simulink model "qs3_dqn_swingup_v4_ctrl"  (R2025b)
settings: Solver=ode1  StartTime=0.0  StopTime=inf  FixedStep=0.002  RelTol=1e-3  AbsTol=1e-6  EnableMultiTasking=on
undefined symbols (not defined in the file): HIL, qc_get_step_size
libraries: quarc_library x3, simulink_extras x3
settings Model: SimulationMode=external  ExtModeTrigDuration=5000  Creator=MLevis  LastModifiedBy=CPB0
settings SolverCC: AutoScaleAbsTol=off  AlgebraicLoopSolver=TrustRegion  PositivePriorityOrder=on
settings DataIOCC: SaveFormat=Array  SignalLoggingSaveFormat=ModelDataLogs  ReturnWorkspaceOutputs=off
settings OptimizationCC: BlockReduction=off  BooleanDataType=off  OptimizeBlockIOStorage=off  BufferReuse=off  GlobalBufferReuse=off  ExpressionFolding=off  ExpressionDepthLimit=2147483647.0  LocalBlockOutputs=off  InitFltsAndDblsToZero=on  OptimizeDataStoreBuffers=off  BusAssignmentInplaceUpdate=off
settings DebuggingCC: SaveWithParameterizedLinksMsg=none  UnderspecifiedInitializationDetection=Classic  MergeDetectMultiDrivingBlocksExec=none  SignalResolutionControl=TryResolveAllWithWarning  MultiTaskDSMMsg=warning  MultiTaskCondExecSysMsg=none  FcnCallInpInsideContextMsg=warning  UnconnectedInputMsg=warning  UnconnectedOutputMsg=warning  UnconnectedLineMsg=warning  StateNameClashWarn=warning  SFUnexpectedBacktrackingDiag=warning  SFNoUnconditionalDefaultTransitionDiag=warning  SFExecutionAtInitializationDiag=none  ArithmeticOperatorsInVariantConditions=warning
settings HardwareCC: TargetHWDeviceType=32-bit Generic
settings ModelReferenceCC: EnableRefExpFcnMdlSchedulingChecks=on  PropagateSignalLabelsOutOfModel=off
settings SFSimCC: SimUseLocalCustomCode=off  CustomCodeUndefinedFunction=UseInterfaceOnly
settings RTWCC: SystemTargetFile=quarc_win64.tlc  TemplateMakefile=quarc_default_tmf  RTWUseLocalCustomCode=off  Toolchain=QUARC win64 | nmake (64-bit Windows)  BuildConfiguration=Faster Runs  GPUComputeCapability=3.5  Description=QUARC Win64 Target Using Toolchain
settings CodeAppCC: StateflowObjectComments=on
settings STFCustomTargetCC: SystemTargetFile=quarc_win64.tlc  UseToolchainInfoCompliant=on
settings GRTTargetCC: ExtMode=on  ExtModeMexFile=quarc_comm  TargetLangStandard=C89/C90 (ANSI)  ParMdlRefBuildCompliant=off  CompOptLevelCompliant=off  CombineOutputUpdateFcns=off  MatFileLogging=off  CPPClassGenCompliant=off  GRTInterface=on
settings ConfigComp: CovMetricSettings=dw  CovSaveCumulativeToWorkspaceVar=on  CovSaveSingleToWorkspaceVar=on  CovExternalEMLEnable=off  CovSFcnEnable=off

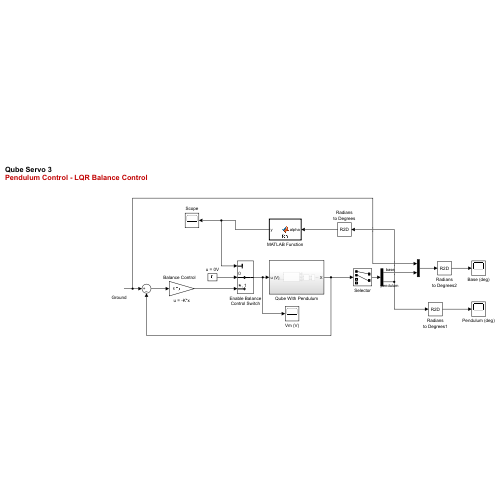
[thumbnail: Simulink's stored preview of the top-level diagram]
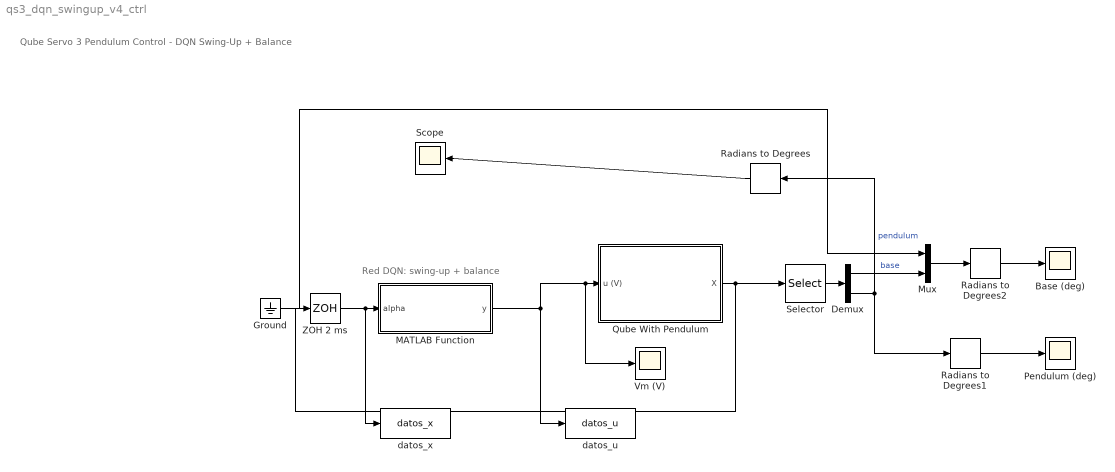
== system qs3_dqn_swingup_v4_ctrl ==
  note: Qube Servo 3
      | Pendulum Control - DQN Swing-Up + Balance
  note: Red DQN: swing-up + balance
  Base (deg) : Scope
      settings: ActiveDisplayYMinimum=-60  ActiveDisplayYMaximum=60
  Demux : Demux  Outputs=2
  Ground : Ground
  MATLAB Function : MATLAB Function  TreatAsAtomicUnit=on
  Mux : Mux  Inputs=2
  Pendulum (deg) : Scope
      settings: ActiveDisplayYMinimum=-224.93408203125  ActiveDisplayYMaximum=224.40673828125  DataLoggingVariableName=ScopeData2
  Qube With Pendulum : Subsystem
  Radians to Degrees : simulink_extras/Transformations/Radians to Degrees
  Radians to Degrees1 : simulink_extras/Transformations/Radians to Degrees
  Radians to Degrees2 : simulink_extras/Transformations/Radians to Degrees
  Scope : Scope
      settings: ActiveDisplayYMinimum=0.9  ActiveDisplayYMaximum=1.1  DataLoggingVariableName=ScopeData3
  Selector : Selector  InputPortWidth=4  IndexOptions=Index vector (dialog)  Indices=[1 2]  OutputSizes=1
  Vm (V) : Scope
      settings: ActiveDisplayYMinimum=-5  ActiveDisplayYMaximum=5
  ZOH 2 ms : ZeroOrderHold  SampleTime=0.002
  datos_x : ToWorkspace  VariableName=datos_x  SampleTime=0.002  SaveFormat=Structure With Time
  datos_u : ToWorkspace  VariableName=datos_u  SampleTime=0.002  SaveFormat=Structure With Time
  wires:
  Demux/1 -> Mux/2  "base"
  Demux/2 -> Radians to Degrees1/1, Radians to Degrees/1  "pendulum"
  Selector/1 -> Demux/1
  Qube With Pendulum/1(X) -> Selector/1, ZOH 2 ms/1
  Mux/1 -> Radians to Degrees2/1
  Radians to Degrees1/1 -> Pendulum (deg)/1
  Radians to Degrees2/1 -> Base (deg)/1
  Ground/1 -> Mux/1
  ZOH 2 ms/1 -> MATLAB Function/1(alpha), datos_x/1
  MATLAB Function/1(y) -> Vm (V)/1, Qube With Pendulum/1("u (V) "), datos_u/1
  Radians to Degrees/1 -> Scope/1

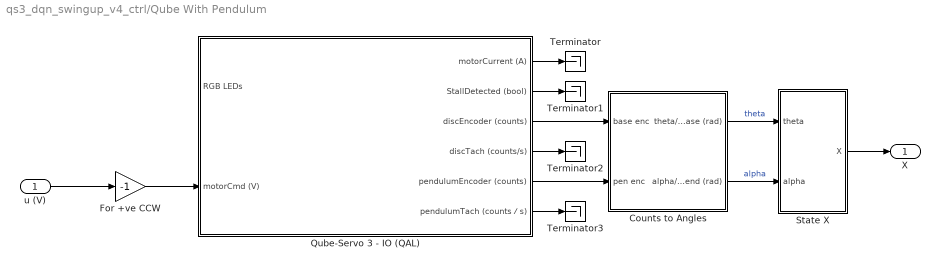
== system qs3_dqn_swingup_v4_ctrl/Qube With Pendulum ==
  "u (V) " : Inport
  Counts to Angles : Subsystem
  For +ve CCW : Gain  Gain=-1
  Qube-Servo 3 - IO (QAL) : Subsystem  mask{setup=Hardware, top=Pendulum}
      mask prompts: setup "Qube-Servo Setup:"; top "Qube Add-On:"
      mask help:
      | This subsystem provides the core and basic I/O capabilities to read data from and write data to the Qube-Servo 3 using the Quanser HIL API. You can write motor commands and LEDs and read motor current, motor stall detection, and base and pendulum encoder and tachometer.
      |
      | The RGB LEDs command is a 3x1 vector representing,
      | 1. Red LED
      | 2. Green LED
      | 3. Blue LED
      mask init:
      | % if nothing is connected to LED, we read RED which will always be 0 so
      |     % that the qube can turn green okay. Once something is connected, we
      |     % read all rgb channels
      |     blockPortData=get_param(gcb,'PortConnectivity');
      |     if (blockPortData(1).SrcBlock==-1)
      |         set_param([gcb, '/HIL Write'], 'other_channels', '[11000]');
      |     else
      |         set_param([gcb, '/HIL Write'], 'other_channels', '[11000:11002]');
      |     end
      | 
      |     % make sure hil blocks match the hil initialize name
      |     set_param([gcb, '/HIL Write'], 'object_name', get_param([gcb, '/HIL Initialize'], 'object_name'));
      |     set_param([gcb, '/HIL Read Timebase'], 'object_name', get_param([gcb, '/HIL Initialize'], 'object_name'));
      |     
      |     % make sure board specific options for qube are always set
      |     set_param([gcb, '/HIL Initialize'], 'board_options', 'deadband_compensation=0.3;pwm_en=0;enc0_velocity=3.0;enc1_velocity=3.0;min_diode_compensation=0.3;max_diode_compensation=1.5');
      |     
      |     % differentiate between hardware and software qubes. Make sure that if
      |     % its hardware, we read both pendulum and disc encoder and tach, even if not
      |     % needed. Hil initialize does not get an ip and port combo. Hil read
      |     % timebase advanced options are set to defaults. 
      |     if strcmp(get_param(gcb, 'setup'), 'Hardware')
      |         set_param([gcb, '/HIL Read Timebase'], 'other_channels', '[14000:14001]');
      |         % set for hardware
      |         set_param([gcb, '/HIL Initialize'], 'board_number', '0');
      |         set_param([gcb, '/HIL Read Timebase'], 'overflow_mode', 'Error on overflow');
      |         set_param([gcb, '/HIL Read Timebase'], 'samples_in_buffer', 'max(ceil(1/qc_get_step_size), 1)');
      |         set_param([gcb, '/HIL Write'], 'active', 'OFF');
      |     % if the qube is virtual, the hil read advanced board specific options
      |     % get set to the correct parameters for virtual cars. 
      |     else
      |         set_param([gcb, '/HIL Read Timebase'], 'overflow_mode', 'Synchronize (for simulated cards only)');
      |         set_param([gcb, '/HIL Read Timebase'], 'samples_in_buffer', '1');
      |         set_param([gcb, '/HIL Write'], 'active', 'ON');
      |     end
      | 
      |     % if set up tach ports for virtual disc vs pendulum. Virtual disc does not support the existence of
      |     % pendulum tach. Also sets up ip and portnumber in the hil initialize. 
      |     if strcmp(get_param(gcb, 'setup'), 'Virtual') && strcmp(get_param(gcb, 'top'), 'Disc')
      |         set_param([gcb, '/HIL Initialize'], 'board_number', '0@tcpip://localhost:18922');
      |         
      |     elseif strcmp(get_param(gcb, 'setup'), 'Virtual') && strcmp(get_param(gcb, 'top'), 'Pendulum')
      |         set_param([gcb, '/HIL Initialize'], 'board_number', '0@tcpip://localhost:18923');
      |         set_param([gcb, '/HIL Read Timebase'], 'other_channels', '[14000:14001]');
      |     end 
      | 
      |     pendulum_encoder_name = 'pendulumEncoder (counts)';
      |     pendulum_encoder = [gcb,'/',pendulum_encoder_name];
      |     
      |     pendulum_tach_name = 'pendulumTach (counts／s)';
      |     pendulum_tach = [gcb,'/',pendulum_tach_name];
      |     
      |     timebase_name = 'HIL Read Timebase';
      |     
      |     % create pendulum encoder and pendulum tach ports and connections if
      |     % needed. Delete them if using the disc. 
      |     if strcmp(get_param(gcb, 'top'), 'Pendulum')
      |         if isempty(find_system(gcbh,'LookUnderMasks','all','Name',pendulum_encoder_name))
      |             add_block('built-in/Outport',pendulum_encoder, 'Port','5','Position',[1050,568,1080,582]);
      |             add_line(gcbh,[timebase_name,'/3'],[pendulum_encoder_name,'/1'],'autorouting','on');
      |         end
      |         if isempty(find_system(gcbh,'LookUnderMasks','all','Name',pendulum_tach_name))
      |             add_block('built-in/Outport',pendulum_tach, 'Port','6','Position',[1050, 603, 1080,617]);
      |             add_line(gcbh,[timebase_name,'/6'],[pendulum_tach_name,'/1'],'autorouting','on');
      |         end 
      |     
      |     else
      |         if ~isempty(find_system(gcbh,'LookUnderMasks','all','Name',pendulum_encoder_name))
      |             delete_line(gcbh,[timebase_name,'/3'],[pendulum_encoder_name,'/1']);
      |             delete_block(pendulum_encoder);
      |         end
      |         if ~isempty(find_system(gcbh,'LookUnderMasks','all','Name',pendulum_tach_name))
      |             delete_line(gcbh,[timebase_name,'/6'],[pendulum_tach_name,'/1']);
      |             delete_block(pendulum_tach);
      |         end 
      |     end
      | 
      |     if strcmp(get_param(gcb, 'setup'), 'Virtual') && strcmp(get_param(gcb, 'top'), 'Disc')
      |         set_param([gcb, '/HIL Read Timebase'], 'other_channels', '[14000]');
      |     end
      settings: CopyFcn=set_param(gcbh,'LinkStatus','none');
      mask TypeOptions setup: Hardware | Virtual
      mask TypeOptions top: Disc | Pendulum
      mask Display:
      | ud = get_param(gcb,'UserData');
      | if (strcmp(get_param(gcb, 'top'), 'Disc') && strcmp(get_param(gcb, 'setup'), 'Hardware'))
      |     image(ud.hardwareDisc);
      | elseif (strcmp(get_param(gcb, 'top'), 'Pendulum') && strcmp(get_param(gcb, 'setup'), 'Hardware'))
      |     image(ud.hardwarePendulum);
      | elseif (strcmp(get_param(gcb, 'top'), 'Disc') && strcmp(get_param(gcb, 'setup'), 'Virtual'))
      |     image(ud.virtualDisc);
      | else
      |     image(ud.virtualPendulum);
      | end
      | 
      | text(.3,.05,'Qube-Servo 3 - IO');
      | 
      | if strcmp(get_param(gcb, 'top'), 'Pendulum')
      |     port_label('input', 1, 'RGB LEDs (%)');
      |     port_label('input', 2, 'motorCmd (V)');
      |     port_label('output', 1, 'Motor Current (A)');
      |     port_label('output', 2, 'StallDetected (bool)');
      |     port_label('output', 3, 'baseEncoder (counts)');
      |     port_label('output', 4, 'baseTach (counts/s)');
      |     port_label('output', 5, 'pendulumEncoder (counts)');
      |     port_label('output', 6, 'pendulumTach (counts/s)');
      | 
      | else
      |     port_label('input', 1, 'RGB LEDs (%)');
      |     port_label('input', 2, 'motorCmd (V)');
      |     port_label('output', 1, 'Motor Current (A)');
      |     port_label('output', 2, 'StallDetected (bool)');
      |     port_label('output', 3, 'baseEncoder (counts)');
      |     port_label('output', 4, 'baseTach (counts/s)');
      | end
  State X : Subsystem
  Terminator{,1..3} (4 alike) : Terminator
  X : Outport
  wires:
  Qube-Servo 3 - IO (QAL)/2(StallDetected (bool)) -> Terminator1/1
  For +ve CCW/1 -> Qube-Servo 3 - IO (QAL)/2(motorCmd (V))
  Qube-Servo 3 - IO (QAL)/6(pendulumTach (counts／s)) -> Terminator3/1
  Qube-Servo 3 - IO (QAL)/5(pendulumEncoder (counts)) -> Counts to Angles/2(pen enc)
  Qube-Servo 3 - IO (QAL)/1(motorCurrent (A)) -> Terminator/1
  Qube-Servo 3 - IO (QAL)/3(discEncoder (counts)) -> Counts to Angles/1(base enc)
  Counts to Angles/2(alpha/pend (rad)) -> State X/2(alpha)  "alpha"
  Qube-Servo 3 - IO (QAL)/4(discTach (counts/s)) -> Terminator2/1
  "u (V) "/1 -> For +ve CCW/1
  Counts to Angles/1(theta/base (rad)) -> State X/1(theta)  "theta"
  State X/1(X) -> X/1

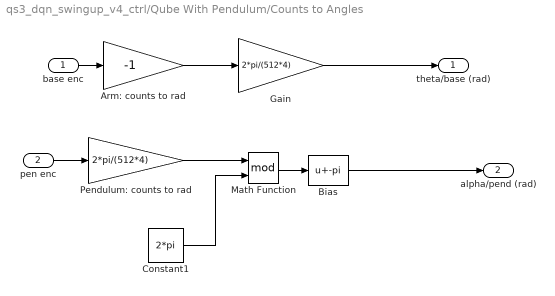
== system qs3_dqn_swingup_v4_ctrl/Qube With Pendulum/Counts to Angles ==
  base enc : Inport
  pen enc : Inport  Port=2
  Arm: counts to rad : Gain  Gain=-1
  Bias : Bias  Bias=-pi  SaturateOnIntegerOverflow=off
  Constant1 : Constant  Value=2*pi
  Gain : Gain  Gain=2*pi/(512*4)
  Math Function : Math  Operator=mod
  Pendulum: counts to rad : Gain  Gain=2*pi/(512*4)
  theta/base (rad) : Outport  VectorParamsAs1DForOutWhenUnconnected=off
  alpha/pend (rad) : Outport  Port=2  VectorParamsAs1DForOutWhenUnconnected=off
  wires:
  base enc/1 -> Arm: counts to rad/1
  pen enc/1 -> Pendulum: counts to rad/1
  Arm: counts to rad/1 -> Gain/1
  Pendulum: counts to rad/1 -> Math Function/1
  Constant1/1 -> Math Function/2
  Math Function/1 -> Bias/1
  Bias/1 -> alpha/pend (rad)/1
  Gain/1 -> theta/base (rad)/1

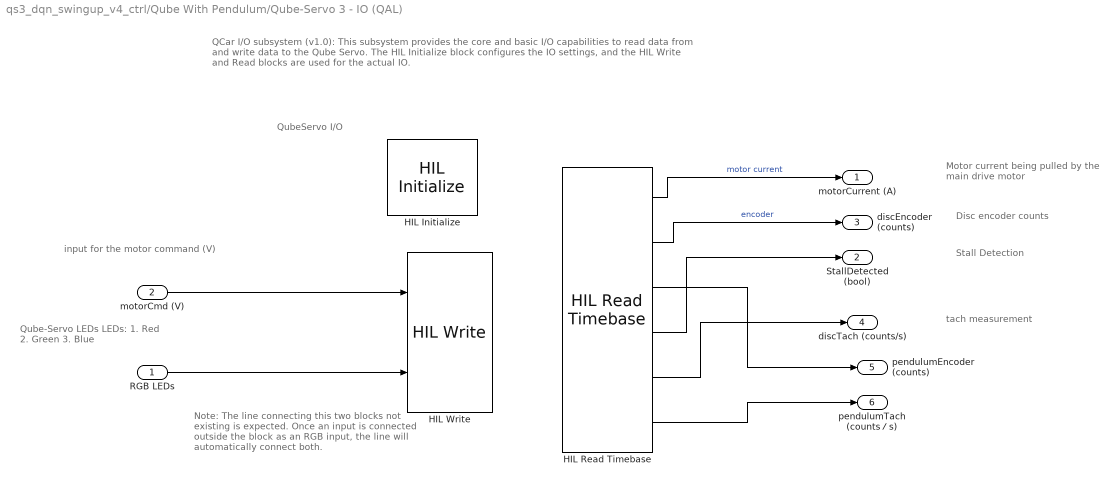
== system qs3_dqn_swingup_v4_ctrl/Qube With Pendulum/Qube-Servo 3 - IO (QAL) ==
  note: Motor current being pulled by the main drive motor
  note: Stall Detection
  note: tach measurement
  note: Disc encoder counts
  note: input for the motor command (V)
  note: QCar I/O subsystem (v1.0):
      |
      | This subsystem provides the core and basic I/O capabilities to read data from and write data to the Qube Servo. The HIL Initialize block configures the IO settings, and the HIL Write and Read blocks are used for the actual IO.
  note: QubeServo I/O
  note: Qube-Servo LEDs
      |
      | LEDs:
      | 1. Red
      | 2. Green
      | 3. Blue
  note: Note: The line connecting this two blocks
      | not existing is expected.
      | Once an input is connected outside the block
      | as an RGB input, the line will automatically
      | connect both.
  RGB LEDs : Inport
  motorCmd (V) : Inport  Port=2
  HIL Initialize : quarc_library/Data Acquisition/Generic/Configuration/HIL Initialize  object_name=HIL-1  board_type=qube_servo3_usb  board_number=0  board_options=deadband_compensation=0.3;pwm_en=0;enc0_velocity=3.0;enc1_velocity=3.0;min_diode_compensation=0.3;max_diode_compensation=1.5  exclusive=off  active=on  hardware_clocks=[0]  clock_modes=[]  initial_clock_frequencies=[]  set_clock_params_at_start=off  set_clock_params_at_switch_in=off  set_clock_frequencies_at_start=off  set_clock_frequencies_at_switch_in=off  analog_input_channels=[0]  analog_input_configurations=[]  analog_input_maximums=3  analog_input_minimums=-3  set_analog_input_params_at_start=off  set_analog_input_params_at_switch_in=off  analog_output_channels=[0]  analog_output_maximums=15  analog_output_minimums=-15  initial_analog_outputs=[0]  final_analog_outputs=[0]  watchdog_analog_outputs=0  set_analog_output_params_at_start=off  set_analog_output_params_at_switch_in=off  set_analog_outputs_at_start=on  set_analog_outputs_at_switch_in=off  set_analog_outputs_at_terminate=on  set_analog_outputs_at_switch_out=off  set_analog_outputs_on_watchdog=on  digital_input_channels=[]  digital_output_channels=[0]  digital_output_configuration=[]  initial_digital_outputs=[1]  final_digital_outputs=[0]  watchdog_digital_outputs=[0]  set_digital_output_params_at_start=off  set_digital_output_params_at_switch_in=off  set_digital_outputs_at_start=on  set_digital_outputs_at_switch_in=off  set_digital_outputs_at_terminate=on  set_digital_outputs_at_switch_out=off  set_digital_outputs_on_watchdog=on  encoder_channels=[0:1]  quadrature=[4]  encoder_filter_frequency=[]  initial_encoder_counts=[0]  set_encoder_params_at_start=off  set_encoder_params_at_switch_in=off  set_encoder_counts_at_start=on  set_encoder_counts_at_switch_in=off  pwm_channels=[]  pwm_modes=[0]  pwm_frequency=23195  pwm_configuration=[1]  pwm_alignment=[0]  pwm_polarity=[1]  pwm_leading_deadband=[0]  pwm_trailing_deadband=[0]  initial_pwm_outputs=[0]  final_pwm_outputs=[0]  watchdog_pwm_outputs=[]  set_pwm_params_at_start=off  set_pwm_params_at_switch_in=off  set_pwm_outputs_at_start=off  set_pwm_outputs_at_switch_in=off  set_pwm_outputs_at_terminate=off  set_pwm_outputs_at_switch_out=off  set_pwm_outputs_on_watchdog=off  other_output_channels=[11000:11002]  initial_other_outputs=[0 1 0]  final_other_outputs=[1 0 0]  watchdog_other_outputs=[0 0 1]  set_other_outputs_at_start=on  set_other_outputs_at_switch_in=off  set_other_outputs_at_terminate=on  set_other_outputs_at_switch_out=off  set_other_outputs_on_watchdog=on
  HIL Read Timebase : quarc_library/Data Acquisition/Generic/Timebases/HIL Read Timebase  object_name=HIL-1  clock=0  analog_channels=[0]  encoder_channels=[0:1]  digital_channels=[1]  other_channels=[14000:14001]  active=on  vector_output=off  data_type_mode=Inherit via back propagation  encoder_data_type=double  digital_data_type=boolean  overflow_mode=Error on overflow  samples_in_buffer=max(ceil(1/qc_get_step_size), 1)
  HIL Write : quarc_library/Data Acquisition/Generic/Immediate I//O/HIL Write  object_name=HIL-1  analog_channels=[0]  pwm_channels=[]  digital_channels=[]  other_channels=[11000]  sample_time=-1  active=off  vector_input=on
  motorCurrent (A) : Outport  VectorParamsAs1DForOutWhenUnconnected=off
  StallDetected (bool) : Outport  Port=2  VectorParamsAs1DForOutWhenUnconnected=off
  discEncoder (counts) : Outport  Port=3  VectorParamsAs1DForOutWhenUnconnected=off
  discTach (counts/s) : Outport  Port=4  VectorParamsAs1DForOutWhenUnconnected=off
  pendulumEncoder (counts) : Outport  Port=5
  pendulumTach (counts／s) : Outport  Port=6
  wires:
  HIL Read Timebase/6 -> pendulumTach (counts／s)/1
  HIL Read Timebase/3 -> pendulumEncoder (counts)/1
  RGB LEDs/1 -> HIL Write/2
  HIL Read Timebase/5 -> discTach (counts/s)/1
  HIL Read Timebase/2 -> discEncoder (counts)/1  "encoder"
  HIL Read Timebase/4 -> StallDetected (bool)/1
  HIL Read Timebase/1 -> motorCurrent (A)/1  "motor current"
  motorCmd (V)/1 -> HIL Write/1

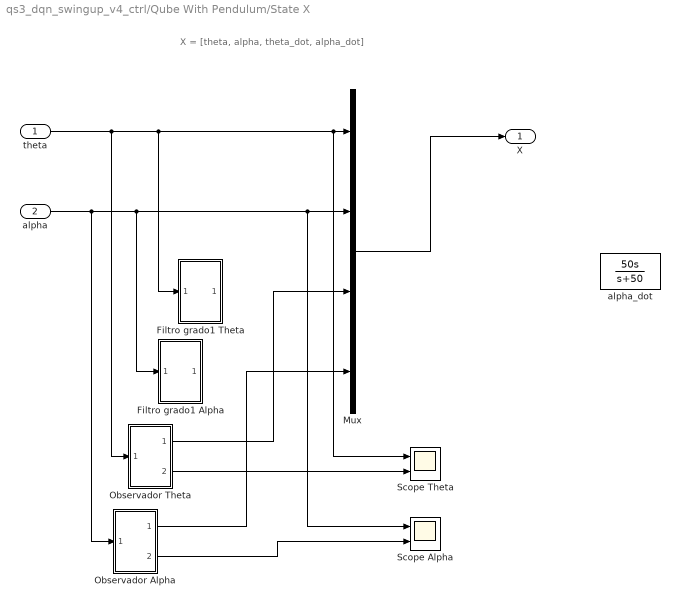
== system qs3_dqn_swingup_v4_ctrl/Qube With Pendulum/State X ==
  note: X = [theta, alpha, theta_dot, alpha_dot]
  theta : Inport
  alpha : Inport  Port=2
  Filtro grado1 Alpha : Subsystem
  Filtro grado1 Theta : Subsystem
  Mux : Mux
  Observador Alpha : Subsystem
  Observador Theta : Subsystem
  Scope Alpha : Scope  NumInputPorts=2
      settings: ActiveDisplayYMinimum=-0.05580573312207239  ActiveDisplayYMaximum=-0.019445990714127122  DataLoggingVariableName=ScopeData5
  Scope Theta : Scope  NumInputPorts=2
      settings: ActiveDisplayYMinimum=-9.2556411891778421  ActiveDisplayYMaximum=9.1728745079339564  DataLoggingVariableName=ScopeData4
  alpha_dot : TransferFcn  Numerator=[50 0]  Denominator=[1 50]
  X : Outport  VectorParamsAs1DForOutWhenUnconnected=off
  wires:
  theta/1 -> Scope Theta/1, Mux/1, Filtro grado1 Theta/1(theta), Observador Theta/1(In1)
  Mux/1 -> X/1
  alpha/1 -> Scope Alpha/1, Mux/2, Filtro grado1 Alpha/1(alpha), Observador Alpha/1(In1)
  Observador Theta/1(dot) -> Mux/3
  Observador Alpha/1(dot) -> Mux/4
  Observador Theta/2(theta) -> Scope Theta/2
  Observador Alpha/2(alfa) -> Scope Alpha/2

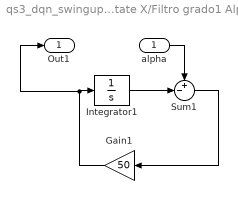
== system qs3_dqn_swingup_v4_ctrl/Qube With Pendulum/State X/Filtro grado1 Alpha ==
  alpha : Inport
  Gain1 : Gain  Gain=50
  Integrator1 : Integrator
  Sum1 : Sum  Inputs=+-|
  Out1 : Outport
  wires:
  Integrator1/1 -> Sum1/2
  Sum1/1 -> Gain1/1
  Gain1/1 -> Out1/1, Integrator1/1
  alpha/1 -> Sum1/1

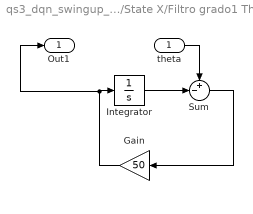
== system qs3_dqn_swingup_v4_ctrl/Qube With Pendulum/State X/Filtro grado1 Theta ==
  theta : Inport
  Gain : Gain  Gain=50
  Integrator : Integrator
  Sum : Sum  Inputs=+-|
  Out1 : Outport
  wires:
  Sum/1 -> Gain/1
  Integrator/1 -> Sum/2
  Gain/1 -> Out1/1, Integrator/1
  theta/1 -> Sum/1

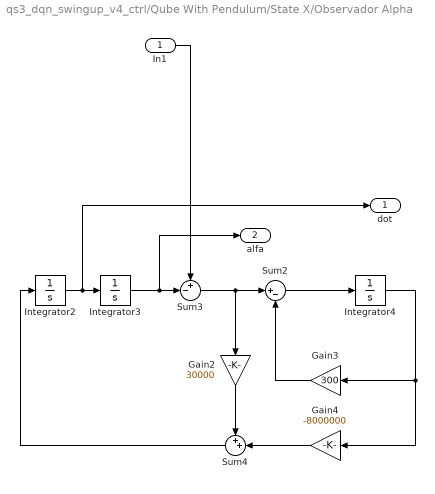
== system qs3_dqn_swingup_v4_ctrl/Qube With Pendulum/State X/Observador Alpha ==
  In1 : Inport
  Gain2 : Gain  Gain=30000
  Gain3 : Gain  Gain=300
  Gain4 : Gain  Gain=-8000000
  Integrator2 : Integrator
  Integrator3 : Integrator
  Integrator4 : Integrator
  Sum2 : Sum  Inputs=|+-
  Sum3 : Sum  Inputs=+-|
  Sum4 : Sum  Inputs=++|
  dot : Outport
  alfa : Outport  Port=2
  wires:
  Integrator2/1 -> dot/1, Integrator3/1
  Integrator4/1 -> Gain3/1, Gain4/1
  Sum2/1 -> Integrator4/1
  In1/1 -> Sum3/1
  Sum4/1 -> Integrator2/1
  Integrator3/1 -> alfa/1, Sum3/2
  Gain2/1 -> Sum4/1
  Sum3/1 -> Gain2/1, Sum2/1
  Gain3/1 -> Sum2/2
  Gain4/1 -> Sum4/2

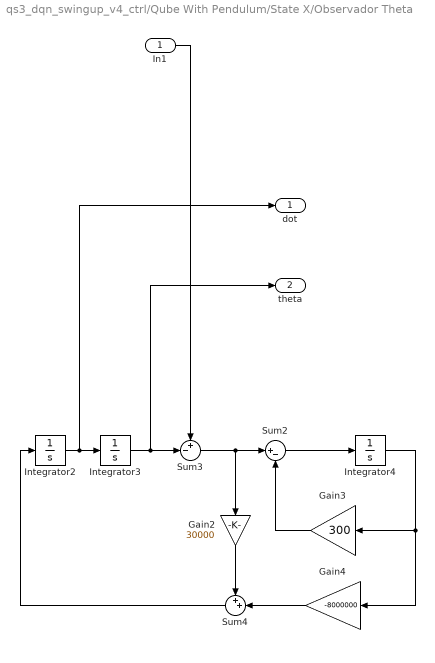
== system qs3_dqn_swingup_v4_ctrl/Qube With Pendulum/State X/Observador Theta ==
  In1 : Inport
  Gain2 : Gain  Gain=30000
  Gain3 : Gain  Gain=300
  Gain4 : Gain  Gain=-8000000
  Integrator2 : Integrator
  Integrator3 : Integrator
  Integrator4 : Integrator
  Sum2 : Sum  Inputs=|+-
  Sum3 : Sum  Inputs=+-|
  Sum4 : Sum  Inputs=++|
  dot : Outport
  theta : Outport  Port=2
  wires:
  Integrator4/1 -> Gain4/1, Gain3/1
  Sum2/1 -> Integrator4/1
  Gain3/1 -> Sum2/2
  Integrator2/1 -> dot/1, Integrator3/1
  Sum3/1 -> Gain2/1, Sum2/1
  Gain2/1 -> Sum4/1
  Integrator3/1 -> theta/1, Sum3/2
  Gain4/1 -> Sum4/2
  Sum4/1 -> Integrator2/1
  In1/1 -> Sum3/1

== matlab function qs3_dqn_swingup_v4_ctrl/MATLAB Function ==
  data: alpha input; y output
function y = fcn(alpha)
%#codegen
% Controlador DQN: swing-up + balance del pendulo.
% La entrada (se llama "alpha" por compatibilidad con el bloque original)
% es la senal X completa de "Qube With Pendulum" (4x1). Salida: voltaje.
% La red se carga al compilar desde dqn_swingup_v4_qube.mat (misma carpeta).
S = coder.load('dqn_swingup_v4_qube.mat', 'red_swingup');
y = dqn_swingup_block(alpha, S.red_swingup);
end

function u = dqn_swingup_block(x, red_swingup)
%DQN_SWINGUP_BLOCK Red DQN que LEVANTA el pendulo (swing-up) y lo MANTIENE
%   arriba. Control inverso: estado medido -> voltaje del motor.  (version 4)
%
%   x          : senal X de "Qube With Pendulum". Solo se usan los angulos de
%                los encoders: x(1) = theta, x(2) = alpha envuelto a (-pi, pi]
%                (0 = arriba, +-pi = colgando).
%   red_swingup: struct guardado en el .mat de la red
%   u          : voltaje del motor (V), YA FILTRADO
%
%   Dentro del bloque:
%   1) Velocidades con el observador de 3er orden del proyecto, en dos
%      versiones (lenta a = 100 y rapida a = 250), usando alpha DESENROLLADO.
%   2) La red decide cada n_hold pasos: un voltaje, o un incremento de voltaje
%      si red_swingup.incremental = 1.
%   3) FILTRO PASA BAJAS de 2.o orden a la salida (filtro_w rad/s, filtro_zeta),
%      integrado con Euler a Ts igual que el bloque continuo con ode1. La red
%      se entreno con este filtro: NO agregar otro filtro despues del bloque.
%
%   Debe ejecutarse cada red_swingup.Ts = 2 ms (ZOH a la entrada).
%   Seguridad: si |theta| > theta_max el voltaje queda en 0 hasta reiniciar.
%#codegen
persistent a_prev a_unw p_o v_o z_o cnt u_cmd f1 f2 apagado
theta = x(1);  alpha = x(2);
if isempty(a_prev)
    a_prev = alpha;  a_unw = alpha;
    p_o = [theta theta; alpha alpha];     % filas: theta, alpha; columnas: lento, rapido
    v_o = zeros(2, 2);  z_o = zeros(2, 2);
    cnt = 0;  u_cmd = 0;  f1 = 0;  f2 = 0;  apagado = false;
end
Ts = red_swingup.Ts;

% --- alpha desenrollado (sin el salto de 2*pi)
d = alpha - a_prev;
d = d - 2*pi*round(d/(2*pi));
a_unw  = a_unw + d;
a_prev = alpha;

% --- observadores de velocidad (Euler a Ts, como ode1)
Lg = [1; 1]*red_swingup.obs_L(:)';
mg = [1; 1]*red_swingup.obs_m(:)';
bg = [1; 1]*red_swingup.obs_beta(:)';
vel = v_o;
e   = [theta theta; a_unw a_unw] - p_o;
p_n = p_o + Ts*v_o;
v_n = v_o + Ts*(Lg.*e + mg.*z_o);
z_n = z_o + Ts*(e - bg.*z_o);
p_o = p_n;  v_o = v_n;  z_o = z_n;

% --- red neuronal: decide cada n_hold pasos
if cnt == 0
    obs = [theta; sin(alpha); cos(alpha); vel(1,1); vel(2,1); vel(1,2); vel(2,2); ...
           u_cmd; f1; f2]./red_swingup.x_scale(:);
    h1 = max(red_swingup.W1*obs + red_swingup.b1(:), 0);
    h2 = max(red_swingup.W2*h1  + red_swingup.b2(:), 0);
    q  = red_swingup.W3*h2 + red_swingup.b3(:);
    [~, i] = max(q);
    if red_swingup.incremental > 0.5
        u_cmd = u_cmd + red_swingup.acciones(i);
    else
        u_cmd = red_swingup.acciones(i);
    end
    u_cmd = min(max(u_cmd, -red_swingup.Vmax), red_swingup.Vmax);
end
cnt = cnt + 1;
if cnt >= red_swingup.n_hold, cnt = 0; end

% --- filtro pasa bajas de 2.o orden: la salida es el estado (como un integrador)
u_f = f1;
w   = red_swingup.filtro_w;
f1n = f1 + Ts*f2;
f2n = f2 + Ts*(w*w*(u_cmd - f1) - 2*red_swingup.filtro_zeta*w*f2);
f1 = f1n;  f2 = f2n;

% --- seguridad: brazo demasiado lejos -> cortar voltaje
if abs(theta) > red_swingup.theta_max, apagado = true; end
if apagado
    u = 0;
else
    u = u_f;
end
end
